simulink model "simple_fuzzy_pid"  (R2025b)
settings: Solver=ode4  StartTime=0.0  StopTime=20  FixedStep=0.01  RelTol=1e-3
InitFcn:
  | fp=fullfile(fileparts(get_param(bdroot,'FileName')),'triangle_pid.fis'); simple_fuzzy_pid_fis=readfis(fp); clear fp;
libraries: fuzblock x1
settings Model: Creator=alosw  LastModifiedBy=alosw

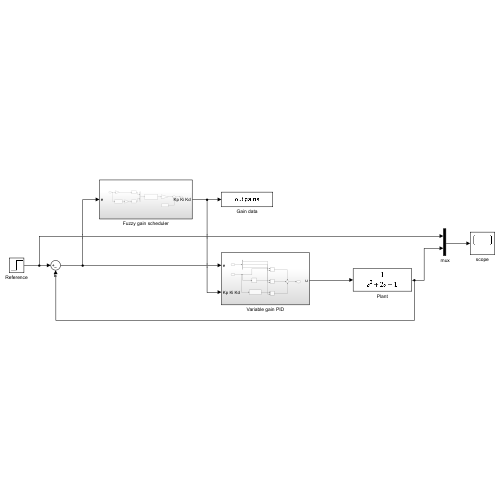
[thumbnail: Simulink's stored preview of the top-level diagram]
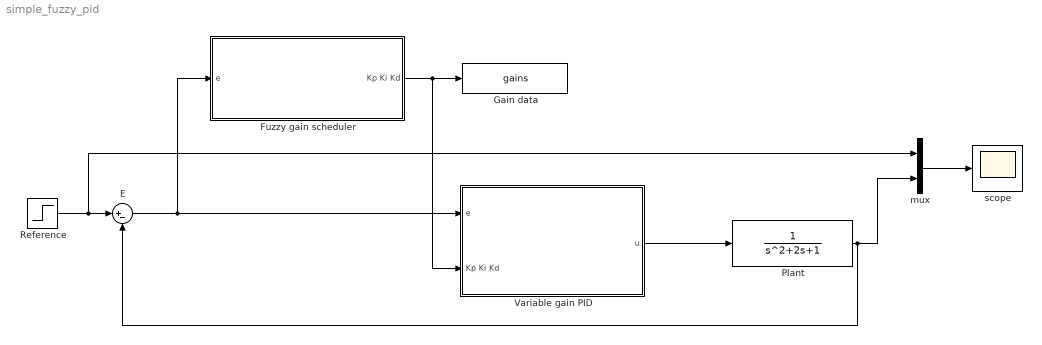
== system simple_fuzzy_pid ==
  " mux" : Mux  Inputs=2
  E : Sum  Inputs=|+-
  Fuzzy gain scheduler : Subsystem
  Gain data : ToWorkspace  VariableName=gains  SaveFormat=Timeseries  SampleTime=-1
  Plant : TransferFcn  Numerator=1
  Reference : Step  SampleTime=0
  Variable gain PID : Subsystem
  scope : Scope
      settings: ActiveDisplayYMinimum=-4.7917876982374583  ActiveDisplayYMaximum=4.3704427415905371
  wires:
  Reference/1 -> E/1, " mux"/1
  E/1 -> Fuzzy gain scheduler/1(e), Variable gain PID/1(e)
  Fuzzy gain scheduler/1(Kp Ki Kd) -> Variable gain PID/2(Kp Ki Kd), Gain data/1
  Variable gain PID/1(u) -> Plant/1
  Plant/1 -> " mux"/2, E/2
  " mux"/1 -> scope/1

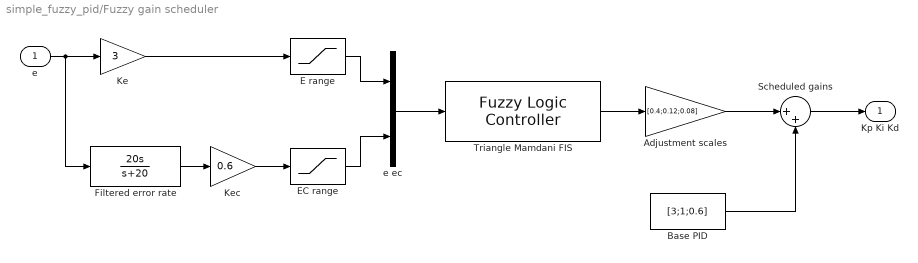
== system simple_fuzzy_pid/Fuzzy gain scheduler ==
  e : Inport
  Adjustment scales : Gain  Gain=[0.4;0.12;0.08]
  Base PID : Constant  Value=[3;1;0.6]
  E range : Saturate  UpperLimit=3  LowerLimit=-3
  EC range : Saturate  UpperLimit=3  LowerLimit=-3
  Filtered error rate : TransferFcn  Numerator=[20 0]  Denominator=[1 20]
  Ke : Gain  Gain=3
  Kec : Gain  Gain=0.6
  Scheduled gains : Sum  Inputs=|++
  Triangle Mamdani FIS : fuzblock/Fuzzy Logic  Controller  FIS=simple_fuzzy_pid_fis  OutputSampleNumber=101  DataType=double  UseLookupTable=off  NumBreakpoints=10  FuzzifiedInputs=off  RuleFiringStrengths=off  RuleOutputs=off  AggregatedOutputs=off  SimulateUsing=Interpreted execution  OutOfRangeInputValueMessage=warning  NoRuleFiredMessage=warning  EmptyOutputFuzzySetMessage=warning
  e ec : Mux  Inputs=2
  Kp Ki Kd : Outport
  wires:
  e/1 -> Filtered error rate/1, Ke/1
  Ke/1 -> E range/1
  Filtered error rate/1 -> Kec/1
  Kec/1 -> EC range/1
  E range/1 -> e ec/1
  EC range/1 -> e ec/2
  e ec/1 -> Triangle Mamdani FIS/1
  Triangle Mamdani FIS/1 -> Adjustment scales/1
  Adjustment scales/1 -> Scheduled gains/1
  Base PID/1 -> Scheduled gains/2
  Scheduled gains/1 -> Kp Ki Kd/1

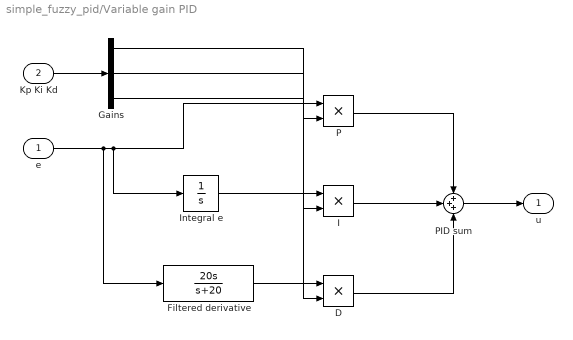
== system simple_fuzzy_pid/Variable gain PID ==
  e : Inport
  Kp Ki Kd : Inport  Port=2
  D : Product
  Filtered derivative : TransferFcn  Numerator=[20 0]  Denominator=[1 20]
  Gains : Demux  Outputs=3
  I : Product
  Integral e : Integrator
  P : Product
  PID sum : Sum  Inputs=+++
  u : Outport
  wires:
  Kp Ki Kd/1 -> Gains/1
  e/1 -> P/1, Integral e/1, Filtered derivative/1
  Integral e/1 -> I/1
  Filtered derivative/1 -> D/1
  Gains/1 -> P/2
  Gains/2 -> I/2
  Gains/3 -> D/2
  P/1 -> PID sum/1
  I/1 -> PID sum/2
  D/1 -> PID sum/3
  PID sum/1 -> u/1
